simulink model "launch_gate_exp"  (R2022b)
settings: Solver=FixedStepDiscrete  StartTime=0.0  StopTime=5  FixedStep=0.001  RelTol=1e-3
InitFcn:
  | if ~exist('P','var') || ~isfield(P,'gate_version'), P=gate_params(launch_tcs_params()); end
model workspace (MAT data in the model file):
  w_2 : Simulink.Parameter (value not decoded)
undefined symbols (not defined in the file): A, a, B, b, C, D, DiscIntNeverNeededParam, Iz, K, k1, K1, k2, K2, L1, L2, m, magnitude, Phi, Sample_time, Steer_Ratio
libraries: simulink x26, slpidlib x13, Solver_SF x1, dsparch4 x1
(part 4 of 7)

== system launch_gate_exp/驱动防滑模块/Subsystem1 ==
  lamda2 : Inport
  p : Inport  Port=2
  i : Inport  Port=3
  b : Inport  Port=4
  Constant : Constant  Value=0.2
  PID Controller : slpidlib/PID Controller  Controller=PI  Form=Parallel  TimeDomain=Discrete-time  UseExternalTs=off  SampleTime=-1  IntegratorMethod=Forward Euler  FilterMethod=Forward Euler  ControllerParametersSource=external  P=5000  I=3000  UseKiTs=off  D=0  N=100  UseFilter=on  TunerSelectOption=Transfer Function Based (PID Tuner App)  InitialConditionSource=internal  InitialConditionForIntegrator=0  InitialConditionForFilter=0  DifferentiatorICPrevScaledInput=0  ExternalReset=none  TrackingMode=off  Kt=1  LimitOutput=on  SatLimitsSource=internal  UpperSaturationLimit=0  LowerSaturationLimit=-30000  LinearizeAsGain=on  AntiWindupMode=clamping  Kb=1  LimitIntegrator=off  UpperIntegratorSaturationLimit=inf  LowerIntegratorSaturationLimit=-inf  POutMin=[]  POutMax=[]  IOutMin=[]  IOutMax=[]  DOutMin=[]  DOutMax=[]  NOutMin=[]  NOutMax=[]  SumOutMin=[]  SumOutMax=[]  SaturationOutMin=[]  SaturationOutMax=[]  PParamMin=[]  PParamMax=[]  IParamMin=[]  IParamMax=[]  DParamMin=[]  DParamMax=[]  NParamMin=[]  NParamMax=[]  KbParamMin=[]  KbParamMax=[]  KtParamMin=[]  KtParamMax=[]  KbOutMin=[]  KbOutMax=[]  KtOutMin=[]  KtOutMax=[]  IntegratorOutMin=[]  IntegratorOutMax=[]  FilterOutMin=[]  FilterOutMax=[]  SumI1OutMin=[]  SumI1OutMax=[]  SumI2OutMin=[]  SumI2OutMax=[]  SumI3OutMin=[]  SumI3OutMax=[]  SumI4OutMin=[]  SumI4OutMax=[]  SumDOutMin=[]  SumDOutMax=[]  DifferentiatorOutMin=[]  DifferentiatorOutMax=[]  FilterDiffOutCoefMin=[]  FilterDiffOutCoefMax=[]  ReciprocalOutMin=[]  ReciprocalOutMax=[]  SumDenOutMin=[]  SumDenOutMax=[]  SumNumOutMin=[]  SumNumOutMax=[]  DivideOutMin=[]  DivideOutMax=[]  UdiffTsProdOutMin=[]  UdiffTsProdOutMax=[]  NTsProdOutMin=[]  NTsProdOutMax=[]  UintegralTsProdOutMin=[]  UintegralTsProdOutMax=[]  UngainTsProdOutMin=[]  UngainTsProdOutMax=[]  ClampingZeroOutDataTypeStr=Inherit: Inherit via back propagation  ClampingZeroOutMin=[]  ClampingZeroOutMax=[]  FilterDenConstantOutDataTypeStr=Inherit: Inherit via back propagation  FilterDenConstantOutMin=[]  FilterDenConstantOutMax=[]  PCopyOutDataTypeStr=Inherit: Inherit via back propagation  PCopyOutMin=[]  PCopyOutMax=[]  NCopyOutDataTypeStr=Inherit: Inherit via back propagation  NCopyOutMin=[]  NCopyOutMax=[]  IntegratorContinuousStateAttributes=''  IntegratorStateMustResolveToSignalObject=off  IntegratorRTWStateStorageClass=Auto  FilterContinuousStateAttributes=''  FilterStateMustResolveToSignalObject=off  FilterRTWStateStorageClass=Auto  ParallelPVariant=ExternalParameters  IdealPVariant=Disabled  IVariant=ExternalParameters  DVariant=Disabled  IntegratorVariant=Discrete  SatVariant=Enabled  AWVariant=DiscClampingParallel  PCopyVariant=Disabled  TRVariant=Disabled  FdbkBlocksVariant=Forward  IdealPFdbkVariant=Disabled  SatFdbkVariant=Disabled  DerivativeFilterVariant=Disabled  NVariant=Disabled  NCopyVariant=Disabled_SignalSpec  FilterICVariant=Disabled  IntegratorICVariant=InternalICs  ExternalResetVariant=Disabled  TRSumVariant=Passthrough  SumFdbkVariant=Disabled  SumVariant=Sum_PI  TsampFilterVariant=InternalTs  TsampNgainVariant=Passthrough  TsampIntegralVariant=Passthrough  ExternalSaturationOutDataTypeStr=Inherit: Same as second input
  Saturation : Saturate  UpperLimit=30000  LowerLimit=-99999
  Sum4 : Sum  Inputs=|+-
  dT1 : Outport
  wires:
  i/1 -> PID Controller/3
  p/1 -> PID Controller/2
  PID Controller/1 -> Saturation/1  "dT1"
  lamda2/1 -> Sum4/2
  Sum4/1 -> PID Controller/1
  Saturation/1 -> dT1/1
  Constant/1 -> Sum4/1

== system launch_gate_exp/驱动防滑模块/Subsystem2 ==
  lamda3 : Inport
  p : Inport  Port=2
  i : Inport  Port=3
  b : Inport  Port=4
  Constant : Constant  Value=0.2
  PID Controller : slpidlib/PID Controller  Controller=PI  Form=Parallel  TimeDomain=Discrete-time  UseExternalTs=off  SampleTime=-1  IntegratorMethod=Forward Euler  FilterMethod=Forward Euler  ControllerParametersSource=external  P=5000  I=3000  UseKiTs=off  D=0  N=100  UseFilter=on  TunerSelectOption=Transfer Function Based (PID Tuner App)  InitialConditionSource=internal  InitialConditionForIntegrator=0  InitialConditionForFilter=0  DifferentiatorICPrevScaledInput=0  ExternalReset=none  TrackingMode=off  Kt=1  LimitOutput=on  SatLimitsSource=internal  UpperSaturationLimit=0  LowerSaturationLimit=-50000  LinearizeAsGain=on  AntiWindupMode=clamping  Kb=1  LimitIntegrator=off  UpperIntegratorSaturationLimit=inf  LowerIntegratorSaturationLimit=-inf  POutMin=[]  POutMax=[]  IOutMin=[]  IOutMax=[]  DOutMin=[]  DOutMax=[]  NOutMin=[]  NOutMax=[]  SumOutMin=[]  SumOutMax=[]  SaturationOutMin=[]  SaturationOutMax=[]  PParamMin=[]  PParamMax=[]  IParamMin=[]  IParamMax=[]  DParamMin=[]  DParamMax=[]  NParamMin=[]  NParamMax=[]  KbParamMin=[]  KbParamMax=[]  KtParamMin=[]  KtParamMax=[]  KbOutMin=[]  KbOutMax=[]  KtOutMin=[]  KtOutMax=[]  IntegratorOutMin=[]  IntegratorOutMax=[]  FilterOutMin=[]  FilterOutMax=[]  SumI1OutMin=[]  SumI1OutMax=[]  SumI2OutMin=[]  SumI2OutMax=[]  SumI3OutMin=[]  SumI3OutMax=[]  SumI4OutMin=[]  SumI4OutMax=[]  SumDOutMin=[]  SumDOutMax=[]  DifferentiatorOutMin=[]  DifferentiatorOutMax=[]  FilterDiffOutCoefMin=[]  FilterDiffOutCoefMax=[]  ReciprocalOutMin=[]  ReciprocalOutMax=[]  SumDenOutMin=[]  SumDenOutMax=[]  SumNumOutMin=[]  SumNumOutMax=[]  DivideOutMin=[]  DivideOutMax=[]  UdiffTsProdOutMin=[]  UdiffTsProdOutMax=[]  NTsProdOutMin=[]  NTsProdOutMax=[]  UintegralTsProdOutMin=[]  UintegralTsProdOutMax=[]  UngainTsProdOutMin=[]  UngainTsProdOutMax=[]  ClampingZeroOutDataTypeStr=Inherit: Inherit via back propagation  ClampingZeroOutMin=[]  ClampingZeroOutMax=[]  FilterDenConstantOutDataTypeStr=Inherit: Inherit via back propagation  FilterDenConstantOutMin=[]  FilterDenConstantOutMax=[]  PCopyOutDataTypeStr=Inherit: Inherit via back propagation  PCopyOutMin=[]  PCopyOutMax=[]  NCopyOutDataTypeStr=Inherit: Inherit via back propagation  NCopyOutMin=[]  NCopyOutMax=[]  IntegratorContinuousStateAttributes=''  IntegratorStateMustResolveToSignalObject=off  IntegratorRTWStateStorageClass=Auto  FilterContinuousStateAttributes=''  FilterStateMustResolveToSignalObject=off  FilterRTWStateStorageClass=Auto  ParallelPVariant=ExternalParameters  IdealPVariant=Disabled  IVariant=ExternalParameters  DVariant=Disabled  IntegratorVariant=Discrete  SatVariant=Enabled  AWVariant=DiscClampingParallel  PCopyVariant=Disabled  TRVariant=Disabled  FdbkBlocksVariant=Forward  IdealPFdbkVariant=Disabled  SatFdbkVariant=Disabled  DerivativeFilterVariant=Disabled  NVariant=Disabled  NCopyVariant=Disabled_SignalSpec  FilterICVariant=Disabled  IntegratorICVariant=InternalICs  ExternalResetVariant=Disabled  TRSumVariant=Passthrough  SumFdbkVariant=Disabled  SumVariant=Sum_PI  TsampFilterVariant=InternalTs  TsampNgainVariant=Passthrough  TsampIntegralVariant=Passthrough  ExternalSaturationOutDataTypeStr=Inherit: Same as second input
  Saturation : Saturate  UpperLimit=30000  LowerLimit=-99999
  Sum4 : Sum  Inputs=|+-
  dT1 : Outport
  wires:
  Sum4/1 -> PID Controller/1
  lamda3/1 -> Sum4/2
  PID Controller/1 -> Saturation/1  "dT1"
  p/1 -> PID Controller/2
  i/1 -> PID Controller/3
  Saturation/1 -> dT1/1
  Constant/1 -> Sum4/1

== system launch_gate_exp/驱动防滑模块/Subsystem3 ==
  lamda4 : Inport
  p : Inport  Port=2
  i : Inport  Port=3
  b : Inport  Port=4
  Constant : Constant  Value=0.2
  PID Controller : slpidlib/PID Controller  Controller=PI  Form=Parallel  TimeDomain=Discrete-time  UseExternalTs=off  SampleTime=-1  IntegratorMethod=Forward Euler  FilterMethod=Forward Euler  ControllerParametersSource=external  P=5000  I=3000  UseKiTs=off  D=0  N=100  UseFilter=on  TunerSelectOption=Transfer Function Based (PID Tuner App)  InitialConditionSource=internal  InitialConditionForIntegrator=0  InitialConditionForFilter=0  DifferentiatorICPrevScaledInput=0  ExternalReset=none  TrackingMode=off  Kt=1  LimitOutput=on  SatLimitsSource=internal  UpperSaturationLimit=0  LowerSaturationLimit=-50000  LinearizeAsGain=on  AntiWindupMode=clamping  Kb=1  LimitIntegrator=off  UpperIntegratorSaturationLimit=inf  LowerIntegratorSaturationLimit=-inf  POutMin=[]  POutMax=[]  IOutMin=[]  IOutMax=[]  DOutMin=[]  DOutMax=[]  NOutMin=[]  NOutMax=[]  SumOutMin=[]  SumOutMax=[]  SaturationOutMin=[]  SaturationOutMax=[]  PParamMin=[]  PParamMax=[]  IParamMin=[]  IParamMax=[]  DParamMin=[]  DParamMax=[]  NParamMin=[]  NParamMax=[]  KbParamMin=[]  KbParamMax=[]  KtParamMin=[]  KtParamMax=[]  KbOutMin=[]  KbOutMax=[]  KtOutMin=[]  KtOutMax=[]  IntegratorOutMin=[]  IntegratorOutMax=[]  FilterOutMin=[]  FilterOutMax=[]  SumI1OutMin=[]  SumI1OutMax=[]  SumI2OutMin=[]  SumI2OutMax=[]  SumI3OutMin=[]  SumI3OutMax=[]  SumI4OutMin=[]  SumI4OutMax=[]  SumDOutMin=[]  SumDOutMax=[]  DifferentiatorOutMin=[]  DifferentiatorOutMax=[]  FilterDiffOutCoefMin=[]  FilterDiffOutCoefMax=[]  ReciprocalOutMin=[]  ReciprocalOutMax=[]  SumDenOutMin=[]  SumDenOutMax=[]  SumNumOutMin=[]  SumNumOutMax=[]  DivideOutMin=[]  DivideOutMax=[]  UdiffTsProdOutMin=[]  UdiffTsProdOutMax=[]  NTsProdOutMin=[]  NTsProdOutMax=[]  UintegralTsProdOutMin=[]  UintegralTsProdOutMax=[]  UngainTsProdOutMin=[]  UngainTsProdOutMax=[]  ClampingZeroOutDataTypeStr=Inherit: Inherit via back propagation  ClampingZeroOutMin=[]  ClampingZeroOutMax=[]  FilterDenConstantOutDataTypeStr=Inherit: Inherit via back propagation  FilterDenConstantOutMin=[]  FilterDenConstantOutMax=[]  PCopyOutDataTypeStr=Inherit: Inherit via back propagation  PCopyOutMin=[]  PCopyOutMax=[]  NCopyOutDataTypeStr=Inherit: Inherit via back propagation  NCopyOutMin=[]  NCopyOutMax=[]  IntegratorContinuousStateAttributes=''  IntegratorStateMustResolveToSignalObject=off  IntegratorRTWStateStorageClass=Auto  FilterContinuousStateAttributes=''  FilterStateMustResolveToSignalObject=off  FilterRTWStateStorageClass=Auto  ParallelPVariant=ExternalParameters  IdealPVariant=Disabled  IVariant=ExternalParameters  DVariant=Disabled  IntegratorVariant=Discrete  SatVariant=Enabled  AWVariant=DiscClampingParallel  PCopyVariant=Disabled  TRVariant=Disabled  FdbkBlocksVariant=Forward  IdealPFdbkVariant=Disabled  SatFdbkVariant=Disabled  DerivativeFilterVariant=Disabled  NVariant=Disabled  NCopyVariant=Disabled_SignalSpec  FilterICVariant=Disabled  IntegratorICVariant=InternalICs  ExternalResetVariant=Disabled  TRSumVariant=Passthrough  SumFdbkVariant=Disabled  SumVariant=Sum_PI  TsampFilterVariant=InternalTs  TsampNgainVariant=Passthrough  TsampIntegralVariant=Passthrough  ExternalSaturationOutDataTypeStr=Inherit: Same as second input
  Saturation : Saturate  UpperLimit=30000  LowerLimit=-99999
  Sum4 : Sum  Inputs=|+-
  dT1 : Outport
  wires:
  i/1 -> PID Controller/3
  p/1 -> PID Controller/2
  PID Controller/1 -> Saturation/1  "dT1"
  lamda4/1 -> Sum4/2
  Sum4/1 -> PID Controller/1
  Saturation/1 -> dT1/1
  Constant/1 -> Sum4/1

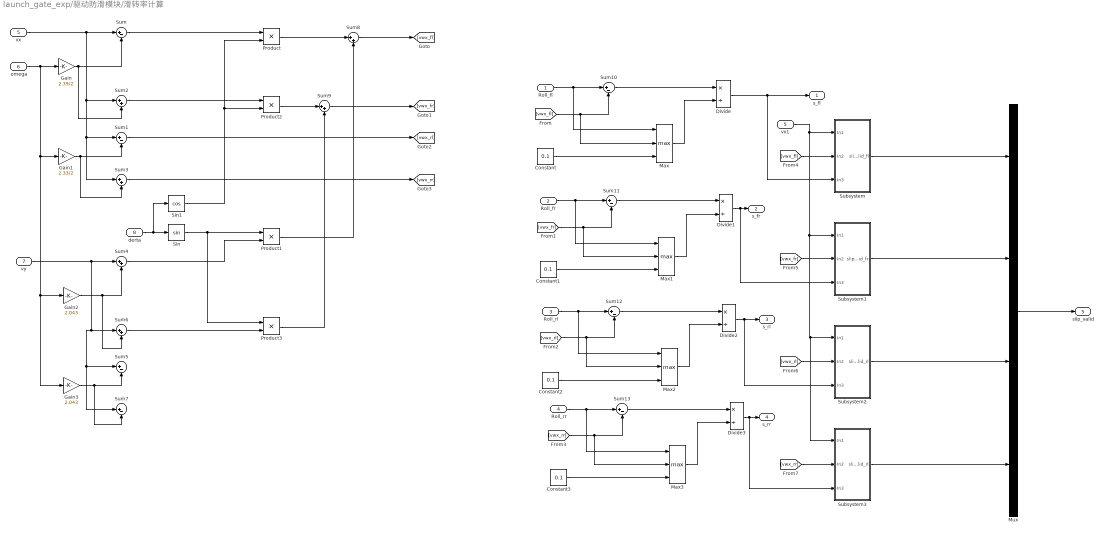
== system launch_gate_exp/驱动防滑模块/滑转率计算 ==
  Roll_fl : Inport
  Roll_fr : Inport  Port=2
  Roll_rl : Inport  Port=3
  Roll_rr : Inport  Port=4
  vx : Inport  Port=5
  omega : Inport  Port=6
  vy : Inport  Port=7
  derta : Inport  Port=8
  Constant{,1..3} (4 alike) : Constant  Value=0.1
  Divide{,1..3} (4 alike) : Product  Inputs=*/
  Gain : Gain  Gain=2.39/2
  Gain1 : Gain  Gain=2.33/2
  Gain2 : Gain  Gain=2.043
  Gain3 : Gain  Gain=2.043
  Max{,1..3} (4 alike) : MinMax  Function=max  Inputs=3
  Mux : Mux
  Product{,1..3} (4 alike) : Product
  Sin : Trigonometry
  Sin1 : Trigonometry  Operator=cos
  Subsystem : Subsystem
  Subsystem1 : Subsystem
  Subsystem2 : Subsystem
  Subsystem3 : Subsystem
  Sum{,1,5,7,10..13} (8 alike) : Sum  Inputs=|+-
  Sum{2..4,6,8..9} (6 alike) : Sum  Inputs=|++
  vx1 : InportShadow  Port=5
  s_fl : Outport
  s_fr : Outport  Port=2
  s_rl : Outport  Port=3
  s_rr : Outport  Port=4
  slip_valid : Outport  Port=5
  wires:
  vx/1 -> Sum3/1, Sum1/1, Sum2/1, Sum/1
  Gain/1 -> Sum2/2, Sum/2
  Gain1/1 -> Sum3/2, Sum1/2
  Gain3/1 -> Sum5/2, Sum7/2
  Gain2/1 -> Sum4/2, Sum6/2
  omega/1 -> Gain3/1, Gain2/1, Gain1/1, Gain/1
  vy/1 -> Sum4/1, Sum5/1, Sum7/1, Sum6/1
  derta/1 -> Sin1/1, Sin/1
  Sum/1 -> Product/1
  Sin1/1 -> Product2/2, Product/2
  Product/1 -> Sum8/1
  Sin/1 -> Product3/1, Product1/1
  Sum4/1 -> Product1/2
  Product1/1 -> Sum8/2
  Sum8/1 -> [vwx_fl]
  Sum2/1 -> Product2/1
  Product2/1 -> Sum9/1
  Sum6/1 -> Product3/2
  Product3/1 -> Sum9/2
  Sum9/1 -> [vwx_fr]
  Sum1/1 -> [vwx_rl]
  Sum3/1 -> [vwx_rr]
  Roll_fl/1 -> Max/1, Sum10/1
  [vwx_fl] -> Max/2, Sum10/2
  Sum10/1 -> Divide/1
  Constant/1 -> Max/3
  Max/1 -> Divide/2
  Divide/1 -> Subsystem/3(In3), s_fl/1
  Divide1/1 -> Subsystem1/3(In3), s_fr/1
  Max1/1 -> Divide1/2
  Constant1/1 -> Max1/3
  Sum11/1 -> Divide1/1
  [vwx_fr] -> Sum11/2, Max1/2
  Roll_fr/1 -> Sum11/1, Max1/1
  Roll_rl/1 -> Max2/1, Sum12/1
  [vwx_rl] -> Max2/2, Sum12/2
  Sum12/1 -> Divide2/1
  Constant2/1 -> Max2/3
  Max2/1 -> Divide2/2
  Divide2/1 -> Subsystem2/3(In3), s_rl/1
  Divide3/1 -> Subsystem3/3(In3), s_rr/1
  Max3/1 -> Divide3/2
  Constant3/1 -> Max3/3
  Sum13/1 -> Divide3/1
  [vwx_rr] -> Sum13/2, Max3/2
  Roll_rr/1 -> Sum13/1, Max3/1
  vx1/1 -> Subsystem3/1(In1), Subsystem2/1(In1), Subsystem1/1(In1), Subsystem/1(In1)
  [vwx_fl] -> Subsystem/2(In2)
  [vwx_fr] -> Subsystem1/2(In2)
  [vwx_rl] -> Subsystem2/2(In2)
  [vwx_rr] -> Subsystem3/2(In2)
  Subsystem/1(slip_valid_fl) -> Mux/1
  Subsystem1/1(slip_valid_fr) -> Mux/2
  Subsystem2/1(slip_valid_rl) -> Mux/3
  Subsystem3/1(slip_valid_rl) -> Mux/4
  Mux/1 -> slip_valid/1

== system launch_gate_exp/Dugoff轮胎模型/alpha_lamda/alpha ==
  vx : Inport
  vy : Inport  Port=2
  wz : Inport  Port=3
  delta_fl : Inport  Port=4
  delta_fr : Inport  Port=5
  Gain{,1..3} (4 alike) : Gain  Gain=-1
  fl : Subsystem
  fr : Subsystem
  rl : Subsystem
  rr : Subsystem
  alpha_fl : Outport
  alpha_fr : Outport  Port=2
  alpha_rl : Outport  Port=3
  alpha_rr : Outport  Port=4
  wires:
  delta_fr/1 -> fr/4(delta_fr)
  delta_fl/1 -> fl/4(delta_fl)
  vy/1 -> rl/2(vy), fl/2(vy), fr/2(vy), rr/2(vy)
  vx/1 -> rl/1(vx), fl/1(vx), fr/1(vx), rr/1(vx)
  wz/1 -> rl/3(wz), fr/3(wz), rr/3(wz), fl/3(wz)
  fl/1(alpha_fl) -> Gain/1
  Gain/1 -> alpha_fl/1
  rl/1(alpha_rl) -> Gain1/1
  Gain1/1 -> alpha_rl/1
  fr/1(alpha_fr) -> Gain2/1
  Gain2/1 -> alpha_fr/1
  rr/1(alpha_rr) -> Gain3/1
  Gain3/1 -> alpha_rr/1

== system launch_gate_exp/Dugoff轮胎模型/alpha_lamda/lamda ==
  vx : Inport
  vy : Inport  Port=2
  wz : Inport  Port=3
  delta_fl : Inport  Port=4
  delta_fr : Inport  Port=5
  w_fl : Inport  Port=6
  w_fr : Inport  Port=7
  w_rl : Inport  Port=8
  w_rr : Inport  Port=9
  fl : Subsystem
  fr : Subsystem
  rl : Subsystem
  rr : Subsystem
  lamda_fl : Outport
  lamda_fr : Outport  Port=2
  lamda_rl : Outport  Port=3
  lamda_rr : Outport  Port=4
  wires:
  fr/1(lamda_fr) -> lamda_fr/1
  rr/1(lamda_rr) -> lamda_rr/1
  w_rl/1 -> rl/1(w_rl)
  w_rr/1 -> rr/1(w_rr)
  w_fr/1 -> fr/1(w_fr)
  delta_fr/1 -> fr/5(delta_fr)
  delta_fl/1 -> fl/5(delta_fl)
  vy/1 -> fl/4(vy), fr/4(vy)
  vx/1 -> fl/3(vx), fr/3(vx), rr/3(vx), rl/3(vx)
  wz/1 -> fl/2(wz), fr/2(wz), rr/2(wz), rl/2(wz)
  w_fl/1 -> fl/1(w_fl)
  rl/1(lamda_rl) -> lamda_rl/1
  fl/1(lamda_fl) -> lamda_fl/1

== system launch_gate_exp/四轮转矩分配/下层轮胎力执行控制器/右前轮 ==
  FzR1 : Inport
  FxR1 : Inport  Port=2
  FyR1 : Inport  Port=3
  kappa_R1 : Inport  Port=4
  derta : Inport  Port=5
  Gain : Gain  Gain=0.834
  If : If  IfExpression=u1 > 52000  ElseIfExpressions=u1<18000
  If Action Subsystem : Subsystem  TreatAsAtomicUnit=on
  If Action Subsystem1 : Subsystem  TreatAsAtomicUnit=on
  If Action Subsystem2 : Subsystem  TreatAsAtomicUnit=on
  Merge : Merge  Inputs=3
  PID Controller : slpidlib/PID Controller  Controller=PID  Form=Parallel  TimeDomain=Discrete-time  UseExternalTs=off  SampleTime=-1  IntegratorMethod=Forward Euler  FilterMethod=Forward Euler  ControllerParametersSource=internal  P=3500  I=3000  UseKiTs=off  D=0  N=100  UseFilter=on  TunerSelectOption=Transfer Function Based (PID Tuner App)  InitialConditionSource=internal  InitialConditionForIntegrator=0  InitialConditionForFilter=0  DifferentiatorICPrevScaledInput=0  ExternalReset=none  TrackingMode=off  Kt=1  LimitOutput=off  SatLimitsSource=internal  UpperSaturationLimit=inf  LowerSaturationLimit=-inf  LinearizeAsGain=on  AntiWindupMode=none  Kb=1  LimitIntegrator=off  UpperIntegratorSaturationLimit=inf  LowerIntegratorSaturationLimit=-inf  POutMin=[]  POutMax=[]  IOutMin=[]  IOutMax=[]  DOutMin=[]  DOutMax=[]  NOutMin=[]  NOutMax=[]  SumOutMin=[]  SumOutMax=[]  SaturationOutMin=[]  SaturationOutMax=[]  PParamMin=[]  PParamMax=[]  IParamMin=[]  IParamMax=[]  DParamMin=[]  DParamMax=[]  NParamMin=[]  NParamMax=[]  KbParamMin=[]  KbParamMax=[]  KtParamMin=[]  KtParamMax=[]  KbOutMin=[]  KbOutMax=[]  KtOutMin=[]  KtOutMax=[]  IntegratorOutMin=[]  IntegratorOutMax=[]  FilterOutMin=[]  FilterOutMax=[]  SumI1OutMin=[]  SumI1OutMax=[]  SumI2OutMin=[]  SumI2OutMax=[]  SumI3OutMin=[]  SumI3OutMax=[]  SumI4OutMin=[]  SumI4OutMax=[]  SumDOutMin=[]  SumDOutMax=[]  DifferentiatorOutMin=[]  DifferentiatorOutMax=[]  FilterDiffOutCoefMin=[]  FilterDiffOutCoefMax=[]  ReciprocalOutMin=[]  ReciprocalOutMax=[]  SumDenOutMin=[]  SumDenOutMax=[]  SumNumOutMin=[]  SumNumOutMax=[]  DivideOutMin=[]  DivideOutMax=[]  UdiffTsProdOutMin=[]  UdiffTsProdOutMax=[]  NTsProdOutMin=[]  NTsProdOutMax=[]  UintegralTsProdOutMin=[]  UintegralTsProdOutMax=[]  UngainTsProdOutMin=[]  UngainTsProdOutMax=[]  ClampingZeroOutDataTypeStr=Inherit: Inherit via back propagation  ClampingZeroOutMin=[]  ClampingZeroOutMax=[]  FilterDenConstantOutDataTypeStr=Inherit: Inherit via back propagation  FilterDenConstantOutMin=[]  FilterDenConstantOutMax=[]  PCopyOutDataTypeStr=Inherit: Inherit via back propagation  PCopyOutMin=[]  PCopyOutMax=[]  NCopyOutDataTypeStr=Inherit: Inherit via back propagation  NCopyOutMin=[]  NCopyOutMax=[]  IntegratorContinuousStateAttributes=''  IntegratorStateMustResolveToSignalObject=off  IntegratorRTWStateStorageClass=Auto  FilterContinuousStateAttributes=''  FilterStateMustResolveToSignalObject=off  FilterRTWStateStorageClass=Auto  ParallelPVariant=InternalParameters  IdealPVariant=Disabled  IVariant=InternalParameters  DVariant=InternalParameters  IntegratorVariant=Discrete  SatVariant=Disabled  AWVariant=Passthrough  PCopyVariant=Disabled  TRVariant=Disabled  FdbkBlocksVariant=Forward  IdealPFdbkVariant=Disabled  SatFdbkVariant=Disabled  DerivativeFilterVariant=ForwardEulerFilter  NVariant=InternalParameters  NCopyVariant=Disabled  FilterICVariant=InternalICsFilter  IntegratorICVariant=InternalICs  ExternalResetVariant=Disabled  TRSumVariant=Passthrough  SumFdbkVariant=Disabled  SumVariant=Sum_PID  TsampFilterVariant=InternalTs  TsampNgainVariant=Passthrough  TsampIntegralVariant=Passthrough  ExternalSaturationOutDataTypeStr=Inherit: Same as second input
  Product : Product
  Product1 : Product
  Saturation1 : Saturate  UpperLimit=1100*63.52  LowerLimit=0
  Sin : Trigonometry
  Sin1 : Trigonometry  Operator=cos
  Sum : Sum  Inputs=|++
  Sum1 : Sum  Inputs=|+-
  Sum2 : Sum  Inputs=|++
  Torque2 : Scope  NumInputPorts=2
  kappa2 : Scope  NumInputPorts=2
  Out1 : Outport
  wires:
  If Action Subsystem1/1(kappa_d) -> Merge/1
  If Action Subsystem2/1(kappa_d) -> Merge/3
  Product1/1 -> Sum/1
  Gain/1 -> Sum2/2
  Product/1 -> Sum/2
  Sin1/1 -> Product1/2
  If/3 -> If Action Subsystem2/Action
  derta/1 -> Sin/1, Sin1/1
  Sum/1 -> Gain/1
  kappa_R1/1 -> kappa2/2, Sum1/2
  FzR1/1 -> If/1
  If Action Subsystem/1(kappa_d) -> Merge/2
  If/2 -> If Action Subsystem/Action
  FyR1/1 -> Product/1
  Sum2/1 -> Torque2/2, Saturation1/1
  Sin/1 -> Product/2
  FxR1/1 -> If Action Subsystem/1(Fx), If Action Subsystem1/1(Fx), If Action Subsystem2/1(Fx), Product1/1
  If/1 -> If Action Subsystem1/Action
  Saturation1/1 -> Out1/1
  Sum1/1 -> PID Controller/1
  Merge/1 -> kappa2/1, Sum1/1
  PID Controller/1 -> Torque2/1, Sum2/1

== system launch_gate_exp/四轮转矩分配/下层轮胎力执行控制器/右后轮 ==
  FzR2 : Inport
  FxR2 : Inport  Port=2
  kappa_R2 : Inport  Port=3
  Gain : Gain  Gain=0.94
  If : If  IfExpression=u1 > 69000  ElseIfExpressions=u1<35000
  If Action Subsystem : Subsystem  TreatAsAtomicUnit=on
  If Action Subsystem1 : Subsystem  TreatAsAtomicUnit=on
  If Action Subsystem2 : Subsystem  TreatAsAtomicUnit=on
  Merge : Merge  Inputs=3
  PID Controller : slpidlib/PID Controller  Controller=PID  Form=Parallel  TimeDomain=Discrete-time  UseExternalTs=off  SampleTime=-1  IntegratorMethod=Forward Euler  FilterMethod=Forward Euler  ControllerParametersSource=internal  P=3500  I=3000  UseKiTs=off  D=0  N=100  UseFilter=on  TunerSelectOption=Transfer Function Based (PID Tuner App)  InitialConditionSource=internal  InitialConditionForIntegrator=0  InitialConditionForFilter=0  DifferentiatorICPrevScaledInput=0  ExternalReset=none  TrackingMode=off  Kt=1  LimitOutput=off  SatLimitsSource=internal  UpperSaturationLimit=inf  LowerSaturationLimit=-inf  LinearizeAsGain=on  AntiWindupMode=none  Kb=1  LimitIntegrator=off  UpperIntegratorSaturationLimit=inf  LowerIntegratorSaturationLimit=-inf  POutMin=[]  POutMax=[]  IOutMin=[]  IOutMax=[]  DOutMin=[]  DOutMax=[]  NOutMin=[]  NOutMax=[]  SumOutMin=[]  SumOutMax=[]  SaturationOutMin=[]  SaturationOutMax=[]  PParamMin=[]  PParamMax=[]  IParamMin=[]  IParamMax=[]  DParamMin=[]  DParamMax=[]  NParamMin=[]  NParamMax=[]  KbParamMin=[]  KbParamMax=[]  KtParamMin=[]  KtParamMax=[]  KbOutMin=[]  KbOutMax=[]  KtOutMin=[]  KtOutMax=[]  IntegratorOutMin=[]  IntegratorOutMax=[]  FilterOutMin=[]  FilterOutMax=[]  SumI1OutMin=[]  SumI1OutMax=[]  SumI2OutMin=[]  SumI2OutMax=[]  SumI3OutMin=[]  SumI3OutMax=[]  SumI4OutMin=[]  SumI4OutMax=[]  SumDOutMin=[]  SumDOutMax=[]  DifferentiatorOutMin=[]  DifferentiatorOutMax=[]  FilterDiffOutCoefMin=[]  FilterDiffOutCoefMax=[]  ReciprocalOutMin=[]  ReciprocalOutMax=[]  SumDenOutMin=[]  SumDenOutMax=[]  SumNumOutMin=[]  SumNumOutMax=[]  DivideOutMin=[]  DivideOutMax=[]  UdiffTsProdOutMin=[]  UdiffTsProdOutMax=[]  NTsProdOutMin=[]  NTsProdOutMax=[]  UintegralTsProdOutMin=[]  UintegralTsProdOutMax=[]  UngainTsProdOutMin=[]  UngainTsProdOutMax=[]  ClampingZeroOutDataTypeStr=Inherit: Inherit via back propagation  ClampingZeroOutMin=[]  ClampingZeroOutMax=[]  FilterDenConstantOutDataTypeStr=Inherit: Inherit via back propagation  FilterDenConstantOutMin=[]  FilterDenConstantOutMax=[]  PCopyOutDataTypeStr=Inherit: Inherit via back propagation  PCopyOutMin=[]  PCopyOutMax=[]  NCopyOutDataTypeStr=Inherit: Inherit via back propagation  NCopyOutMin=[]  NCopyOutMax=[]  IntegratorContinuousStateAttributes=''  IntegratorStateMustResolveToSignalObject=off  IntegratorRTWStateStorageClass=Auto  FilterContinuousStateAttributes=''  FilterStateMustResolveToSignalObject=off  FilterRTWStateStorageClass=Auto  ParallelPVariant=InternalParameters  IdealPVariant=Disabled  IVariant=InternalParameters  DVariant=InternalParameters  IntegratorVariant=Discrete  SatVariant=Disabled  AWVariant=Passthrough  PCopyVariant=Disabled  TRVariant=Disabled  FdbkBlocksVariant=Forward  IdealPFdbkVariant=Disabled  SatFdbkVariant=Disabled  DerivativeFilterVariant=ForwardEulerFilter  NVariant=InternalParameters  NCopyVariant=Disabled  FilterICVariant=InternalICsFilter  IntegratorICVariant=InternalICs  ExternalResetVariant=Disabled  TRSumVariant=Passthrough  SumFdbkVariant=Disabled  SumVariant=Sum_PID  TsampFilterVariant=InternalTs  TsampNgainVariant=Passthrough  TsampIntegralVariant=Passthrough  ExternalSaturationOutDataTypeStr=Inherit: Same as second input
  Saturation3 : Saturate  UpperLimit=1800*80.4  LowerLimit=0
  Sum1 : Sum  Inputs=|+-
  Sum2 : Sum  Inputs=|++
  Torque4 : Scope  NumInputPorts=2
  kappa4 : Scope  NumInputPorts=2
  Out1 : Outport
  wires:
  If/1 -> If Action Subsystem1/Action
  If/2 -> If Action Subsystem/Action
  If Action Subsystem/1(kappa_d) -> Merge/2
  FzR2/1 -> If/1
  Sum1/1 -> PID Controller/1
  FxR2/1 -> If Action Subsystem2/1(Fx), Gain/1, If Action Subsystem1/1(Fx), If Action Subsystem/1(Fx)
  If/3 -> If Action Subsystem2/Action
  Gain/1 -> Sum2/2
  If Action Subsystem2/1(kappa_d) -> Merge/3
  If Action Subsystem1/1(kappa_d) -> Merge/1
  Saturation3/1 -> Out1/1
  Sum2/1 -> Torque4/2, Saturation3/1
  kappa_R2/1 -> kappa4/2, Sum1/2
  Merge/1 -> kappa4/1, Sum1/1
  PID Controller/1 -> Torque4/1, Sum2/1

== system launch_gate_exp/四轮转矩分配/下层轮胎力执行控制器/左前轮 ==
  FzL1 : Inport
  FxL1 : Inport  Port=2
  FyL1 : Inport  Port=3
  kappa_L1 : Inport  Port=4
  derta : Inport  Port=5
  Gain : Gain  Gain=0.834
  If : If  IfExpression=u1 > 52000  ElseIfExpressions=u1<18000
  If Action Subsystem : Subsystem  TreatAsAtomicUnit=on
  If Action Subsystem1 : Subsystem  TreatAsAtomicUnit=on
  If Action Subsystem2 : Subsystem  TreatAsAtomicUnit=on
  Merge : Merge  Inputs=3
  PID Controller : slpidlib/PID Controller  Controller=PID  Form=Parallel  TimeDomain=Discrete-time  UseExternalTs=off  SampleTime=-1  IntegratorMethod=Forward Euler  FilterMethod=Forward Euler  ControllerParametersSource=internal  P=3500  I=3000  UseKiTs=off  D=0  N=100  UseFilter=on  TunerSelectOption=Transfer Function Based (PID Tuner App)  InitialConditionSource=internal  InitialConditionForIntegrator=0  InitialConditionForFilter=0  DifferentiatorICPrevScaledInput=0  ExternalReset=none  TrackingMode=off  Kt=1  LimitOutput=off  SatLimitsSource=internal  UpperSaturationLimit=inf  LowerSaturationLimit=-inf  LinearizeAsGain=on  AntiWindupMode=none  Kb=1  LimitIntegrator=off  UpperIntegratorSaturationLimit=inf  LowerIntegratorSaturationLimit=-inf  POutMin=[]  POutMax=[]  IOutMin=[]  IOutMax=[]  DOutMin=[]  DOutMax=[]  NOutMin=[]  NOutMax=[]  SumOutMin=[]  SumOutMax=[]  SaturationOutMin=[]  SaturationOutMax=[]  PParamMin=[]  PParamMax=[]  IParamMin=[]  IParamMax=[]  DParamMin=[]  DParamMax=[]  NParamMin=[]  NParamMax=[]  KbParamMin=[]  KbParamMax=[]  KtParamMin=[]  KtParamMax=[]  KbOutMin=[]  KbOutMax=[]  KtOutMin=[]  KtOutMax=[]  IntegratorOutMin=[]  IntegratorOutMax=[]  FilterOutMin=[]  FilterOutMax=[]  SumI1OutMin=[]  SumI1OutMax=[]  SumI2OutMin=[]  SumI2OutMax=[]  SumI3OutMin=[]  SumI3OutMax=[]  SumI4OutMin=[]  SumI4OutMax=[]  SumDOutMin=[]  SumDOutMax=[]  DifferentiatorOutMin=[]  DifferentiatorOutMax=[]  FilterDiffOutCoefMin=[]  FilterDiffOutCoefMax=[]  ReciprocalOutMin=[]  ReciprocalOutMax=[]  SumDenOutMin=[]  SumDenOutMax=[]  SumNumOutMin=[]  SumNumOutMax=[]  DivideOutMin=[]  DivideOutMax=[]  UdiffTsProdOutMin=[]  UdiffTsProdOutMax=[]  NTsProdOutMin=[]  NTsProdOutMax=[]  UintegralTsProdOutMin=[]  UintegralTsProdOutMax=[]  UngainTsProdOutMin=[]  UngainTsProdOutMax=[]  ClampingZeroOutDataTypeStr=Inherit: Inherit via back propagation  ClampingZeroOutMin=[]  ClampingZeroOutMax=[]  FilterDenConstantOutDataTypeStr=Inherit: Inherit via back propagation  FilterDenConstantOutMin=[]  FilterDenConstantOutMax=[]  PCopyOutDataTypeStr=Inherit: Inherit via back propagation  PCopyOutMin=[]  PCopyOutMax=[]  NCopyOutDataTypeStr=Inherit: Inherit via back propagation  NCopyOutMin=[]  NCopyOutMax=[]  IntegratorContinuousStateAttributes=''  IntegratorStateMustResolveToSignalObject=off  IntegratorRTWStateStorageClass=Auto  FilterContinuousStateAttributes=''  FilterStateMustResolveToSignalObject=off  FilterRTWStateStorageClass=Auto  ParallelPVariant=InternalParameters  IdealPVariant=Disabled  IVariant=InternalParameters  DVariant=InternalParameters  IntegratorVariant=Discrete  SatVariant=Disabled  AWVariant=Passthrough  PCopyVariant=Disabled  TRVariant=Disabled  FdbkBlocksVariant=Forward  IdealPFdbkVariant=Disabled  SatFdbkVariant=Disabled  DerivativeFilterVariant=ForwardEulerFilter  NVariant=InternalParameters  NCopyVariant=Disabled  FilterICVariant=InternalICsFilter  IntegratorICVariant=InternalICs  ExternalResetVariant=Disabled  TRSumVariant=Passthrough  SumFdbkVariant=Disabled  SumVariant=Sum_PID  TsampFilterVariant=InternalTs  TsampNgainVariant=Passthrough  TsampIntegralVariant=Passthrough  ExternalSaturationOutDataTypeStr=Inherit: Same as second input
  Product : Product
  Product1 : Product
  Saturation1 : Saturate  UpperLimit=1100*63.52  LowerLimit=0
  Sin : Trigonometry
  Sin1 : Trigonometry  Operator=cos
  Sum : Sum  Inputs=|++
  Sum1 : Sum  Inputs=|+-
  Sum2 : Sum  Inputs=|++
  Torque : Scope  NumInputPorts=2
  kappa : Scope  NumInputPorts=2
  Out1 : Outport
  wires:
  If/1 -> If Action Subsystem1/Action
  FxL1/1 -> Product1/1, If Action Subsystem2/1(Fx), If Action Subsystem1/1(Fx), If Action Subsystem/1(Fx)
  Sin/1 -> Product/2
  Sum2/1 -> Torque/2, Saturation1/1
  FyL1/1 -> Product/1
  If/2 -> If Action Subsystem/Action
  If Action Subsystem/1(kappa_d) -> Merge/2
  FzL1/1 -> If/1
  kappa_L1/1 -> kappa/2, Sum1/2
  Sum1/1 -> PID Controller/1
  Sum/1 -> Gain/1
  derta/1 -> Sin1/1, Sin/1
  If/3 -> If Action Subsystem2/Action
  Sin1/1 -> Product1/2
  Merge/1 -> kappa/1, Sum1/1
  Product/1 -> Sum/2
  Gain/1 -> Sum2/2
  PID Controller/1 -> Torque/1, Sum2/1
  Product1/1 -> Sum/1
  If Action Subsystem2/1(kappa_d) -> Merge/3
  If Action Subsystem1/1(kappa_d) -> Merge/1
  Saturation1/1 -> Out1/1

== system launch_gate_exp/四轮转矩分配/下层轮胎力执行控制器/左后轮 ==
  FzL2 : Inport
  FxL2 : Inport  Port=2
  kappa_L2 : Inport  Port=3
  Gain : Gain  Gain=0.94
  If : If  IfExpression=u1 > 69000  ElseIfExpressions=u1<35000
  If Action Subsystem : Subsystem  TreatAsAtomicUnit=on
  If Action Subsystem1 : Subsystem  TreatAsAtomicUnit=on
  If Action Subsystem2 : Subsystem  TreatAsAtomicUnit=on
  Merge : Merge  Inputs=3
  PID Controller : slpidlib/PID Controller  Controller=PID  Form=Parallel  TimeDomain=Discrete-time  UseExternalTs=off  SampleTime=-1  IntegratorMethod=Forward Euler  FilterMethod=Forward Euler  ControllerParametersSource=internal  P=3500  I=3000  UseKiTs=off  D=0  N=100  UseFilter=on  TunerSelectOption=Transfer Function Based (PID Tuner App)  InitialConditionSource=internal  InitialConditionForIntegrator=0  InitialConditionForFilter=0  DifferentiatorICPrevScaledInput=0  ExternalReset=none  TrackingMode=off  Kt=1  LimitOutput=off  SatLimitsSource=internal  UpperSaturationLimit=inf  LowerSaturationLimit=-inf  LinearizeAsGain=on  AntiWindupMode=none  Kb=1  LimitIntegrator=off  UpperIntegratorSaturationLimit=inf  LowerIntegratorSaturationLimit=-inf  POutMin=[]  POutMax=[]  IOutMin=[]  IOutMax=[]  DOutMin=[]  DOutMax=[]  NOutMin=[]  NOutMax=[]  SumOutMin=[]  SumOutMax=[]  SaturationOutMin=[]  SaturationOutMax=[]  PParamMin=[]  PParamMax=[]  IParamMin=[]  IParamMax=[]  DParamMin=[]  DParamMax=[]  NParamMin=[]  NParamMax=[]  KbParamMin=[]  KbParamMax=[]  KtParamMin=[]  KtParamMax=[]  KbOutMin=[]  KbOutMax=[]  KtOutMin=[]  KtOutMax=[]  IntegratorOutMin=[]  IntegratorOutMax=[]  FilterOutMin=[]  FilterOutMax=[]  SumI1OutMin=[]  SumI1OutMax=[]  SumI2OutMin=[]  SumI2OutMax=[]  SumI3OutMin=[]  SumI3OutMax=[]  SumI4OutMin=[]  SumI4OutMax=[]  SumDOutMin=[]  SumDOutMax=[]  DifferentiatorOutMin=[]  DifferentiatorOutMax=[]  FilterDiffOutCoefMin=[]  FilterDiffOutCoefMax=[]  ReciprocalOutMin=[]  ReciprocalOutMax=[]  SumDenOutMin=[]  SumDenOutMax=[]  SumNumOutMin=[]  SumNumOutMax=[]  DivideOutMin=[]  DivideOutMax=[]  UdiffTsProdOutMin=[]  UdiffTsProdOutMax=[]  NTsProdOutMin=[]  NTsProdOutMax=[]  UintegralTsProdOutMin=[]  UintegralTsProdOutMax=[]  UngainTsProdOutMin=[]  UngainTsProdOutMax=[]  ClampingZeroOutDataTypeStr=Inherit: Inherit via back propagation  ClampingZeroOutMin=[]  ClampingZeroOutMax=[]  FilterDenConstantOutDataTypeStr=Inherit: Inherit via back propagation  FilterDenConstantOutMin=[]  FilterDenConstantOutMax=[]  PCopyOutDataTypeStr=Inherit: Inherit via back propagation  PCopyOutMin=[]  PCopyOutMax=[]  NCopyOutDataTypeStr=Inherit: Inherit via back propagation  NCopyOutMin=[]  NCopyOutMax=[]  IntegratorContinuousStateAttributes=''  IntegratorStateMustResolveToSignalObject=off  IntegratorRTWStateStorageClass=Auto  FilterContinuousStateAttributes=''  FilterStateMustResolveToSignalObject=off  FilterRTWStateStorageClass=Auto  ParallelPVariant=InternalParameters  IdealPVariant=Disabled  IVariant=InternalParameters  DVariant=InternalParameters  IntegratorVariant=Discrete  SatVariant=Disabled  AWVariant=Passthrough  PCopyVariant=Disabled  TRVariant=Disabled  FdbkBlocksVariant=Forward  IdealPFdbkVariant=Disabled  SatFdbkVariant=Disabled  DerivativeFilterVariant=ForwardEulerFilter  NVariant=InternalParameters  NCopyVariant=Disabled  FilterICVariant=InternalICsFilter  IntegratorICVariant=InternalICs  ExternalResetVariant=Disabled  TRSumVariant=Passthrough  SumFdbkVariant=Disabled  SumVariant=Sum_PID  TsampFilterVariant=InternalTs  TsampNgainVariant=Passthrough  TsampIntegralVariant=Passthrough  ExternalSaturationOutDataTypeStr=Inherit: Same as second input
  Saturation3 : Saturate  UpperLimit=1800*80.4  LowerLimit=0
  Sum1 : Sum  Inputs=|+-
  Sum2 : Sum  Inputs=|++
  Torque3 : Scope  NumInputPorts=2
  kappa3 : Scope  NumInputPorts=2
  Out1 : Outport
  wires:
  Saturation3/1 -> Out1/1
  If Action Subsystem1/1(kappa_d) -> Merge/1
  If Action Subsystem2/1(kappa_d) -> Merge/3
  Gain/1 -> Sum2/2
  If/3 -> If Action Subsystem2/Action
  FxL2/1 -> If Action Subsystem/1(Fx), If Action Subsystem1/1(Fx), Gain/1, If Action Subsystem2/1(Fx)
  kappa_L2/1 -> kappa3/2, Sum1/2
  FzL2/1 -> If/1
  If Action Subsystem/1(kappa_d) -> Merge/2
  If/2 -> If Action Subsystem/Action
  If/1 -> If Action Subsystem1/Action
  Sum2/1 -> Torque3/2, Saturation3/1
  Sum1/1 -> PID Controller/1
  Merge/1 -> kappa3/1, Sum1/1
  PID Controller/1 -> Torque3/1, Sum2/1

== system launch_gate_exp/总驱动力矩制定/正常工况_高速衰减防抖/Subsystem1 ==
  v : Inport
  Add : Sum
  Constant : Constant  Value=200
  Constant1 : Constant  Value=50
  Constant2 : Constant  Value=5
  Divide : Product  Inputs=*/
  Gain : Gain  Gain=5000-200
  Sum : Sum  Inputs=|+-
  Out1 : Outport
  wires:
  Add/1 -> Out1/1
  Gain/1 -> Add/2
  Divide/1 -> Gain/1
  Constant2/1 -> Divide/2
  Sum/1 -> Divide/1
  v/1 -> Sum/2
  Constant1/1 -> Sum/1
  Constant/1 -> Add/1

== system launch_gate_exp/总驱动力矩制定/正常工况_高速衰减防抖/高速衰减冻结区 ==
  v : Inport
  Add : Sum
  Constant : Constant  Value=200
  Constant1 : Constant  Value=20
  Constant2 : Constant  Value=2
  Divide : Product  Inputs=*/
  Gain : Gain  Gain=1000-200
  Sum : Sum  Inputs=|+-
  Out1 : Outport
  wires:
  Constant/1 -> Add/1
  Constant1/1 -> Sum/1
  v/1 -> Sum/2
  Sum/1 -> Divide/1
  Constant2/1 -> Divide/2
  Divide/1 -> Gain/1
  Gain/1 -> Add/2
  Add/1 -> Out1/1

== system launch_gate_exp/质心侧偏角估计/Observer/Subsystem ==
  note: yhat[k|k-1]
  L[k] : Inport
  y[k] : Inport  Port=2
  C[k] : Inport  Port=3
  xhat[k|k-1] : Inport  Port=4
  D[k] : Inport  Port=5
  u[k] : Inport  Port=6
  Add : Sum  Inputs=+-
  Add1 : Sum
  C[k]*xhat[k|k-1] : Product  Multiplication=Matrix(*)
  D[k]*u[k] : Product  Multiplication=Matrix(*)
  Matrix Multiply : Product  Multiplication=Matrix(*)
  L*(y[k]-yhat[k|k-1]) : Outport
  wires:
  L[k]/1 -> Matrix Multiply/1
  y[k]/1 -> Add/1
  C[k]/1 -> C[k]*xhat[k|k-1]/1
  xhat[k|k-1]/1 -> C[k]*xhat[k|k-1]/2
  C[k]*xhat[k|k-1]/1 -> Add1/1
  D[k]/1 -> D[k]*u[k]/1
  u[k]/1 -> D[k]*u[k]/2
  D[k]*u[k]/1 -> Add1/2
  Add1/1 -> Add/2
  Add/1 -> Matrix Multiply/2
  Matrix Multiply/1 -> L*(y[k]-yhat[k|k-1])/1

== system launch_gate_exp/质心侧偏角滑模观测器估计/Subsystem/Subsystem ==
  error : Inport
  Abs : Abs  SaturateOnIntegerOverflow=off
  Discrete-Time Integrator : DiscreteIntegrator  SampleTime=-1  ICPrevOutput=DiscIntNeverNeededParam  ICPrevScaledInput=DiscIntNeverNeededParam
  Gain : Gain  Gain=K1
  Gain1 : Gain  Gain=K2
  Product : Product
  Sign : Signum
  Sqrt : Sqrt
  Sum : Sum  Inputs=|++
  v_STA : Outport
  wires:
  error/1 -> Abs/1, Sign/1
  Abs/1 -> Sqrt/1
  Sqrt/1 -> Product/1
  Sign/1 -> Gain1/1, Product/2
  Product/1 -> Gain/1
  Gain1/1 -> Discrete-Time Integrator/1
  Sum/1 -> v_STA/1
  Gain/1 -> Sum/1
  Discrete-Time Integrator/1 -> Sum/2

== system launch_gate_exp/驱动防滑模块/滑转率计算/Subsystem ==
  In1 : Inport
  In2 : Inport  Port=2
  In3 : Inport  Port=3
  Abs : Abs  SaturateOnIntegerOverflow=off
  Constant4 : Constant  Value=0.1
  Constant5 : Constant  Value=0.2
  Constant6 : Constant  Value=-1.2
  Constant7 : Constant  Value=1.2
  Logical Operator : Logic  Inputs=3  AllPortsSameDT=off  OutDataTypeStr=boolean
  Logical Operator1 : Logic  AllPortsSameDT=off  OutDataTypeStr=boolean
  Relational Operator : RelationalOperator  OutDataTypeStr=boolean  RndMeth=Simplest  InputSameDT=off
  Relational Operator1 : RelationalOperator  OutDataTypeStr=boolean  RndMeth=Simplest  InputSameDT=off
  Relational Operator2 : RelationalOperator  Operator=>  OutDataTypeStr=boolean  RndMeth=Simplest  InputSameDT=off
  Relational Operator3 : RelationalOperator  Operator=<  OutDataTypeStr=boolean  RndMeth=Simplest  InputSameDT=off
  slip_valid_fl : Outport
  wires:
  Logical Operator1/1 -> Logical Operator/3
  Constant4/1 -> Relational Operator/2
  Relational Operator/1 -> Logical Operator/1
  Constant7/1 -> Relational Operator3/2
  In3/1 -> Relational Operator3/1, Relational Operator2/1
  Abs/1 -> Relational Operator/1
  Constant5/1 -> Relational Operator1/2
  Relational Operator2/1 -> Logical Operator1/1
  Constant6/1 -> Relational Operator2/2
  In1/1 -> Abs/1
  Relational Operator3/1 -> Logical Operator1/2
  In2/1 -> Relational Operator1/1
  Relational Operator1/1 -> Logical Operator/2
  Logical Operator/1 -> slip_valid_fl/1

== system launch_gate_exp/驱动防滑模块/滑转率计算/Subsystem1 ==
  In1 : Inport
  In2 : Inport  Port=2
  In3 : Inport  Port=3
  Abs : Abs  SaturateOnIntegerOverflow=off
  Constant4 : Constant  Value=0.1
  Constant5 : Constant  Value=0.2
  Constant6 : Constant  Value=-1.2
  Constant7 : Constant  Value=1.2
  Logical Operator : Logic  Inputs=3  AllPortsSameDT=off  OutDataTypeStr=boolean
  Logical Operator1 : Logic  AllPortsSameDT=off  OutDataTypeStr=boolean
  Relational Operator : RelationalOperator  OutDataTypeStr=boolean  RndMeth=Simplest  InputSameDT=off
  Relational Operator1 : RelationalOperator  OutDataTypeStr=boolean  RndMeth=Simplest  InputSameDT=off
  Relational Operator2 : RelationalOperator  Operator=>  OutDataTypeStr=boolean  RndMeth=Simplest  InputSameDT=off
  Relational Operator3 : RelationalOperator  Operator=<  OutDataTypeStr=boolean  RndMeth=Simplest  InputSameDT=off
  slip_valid_fr : Outport
  wires:
  Logical Operator/1 -> slip_valid_fr/1
  Relational Operator1/1 -> Logical Operator/2
  In2/1 -> Relational Operator1/1
  Relational Operator3/1 -> Logical Operator1/2
  In1/1 -> Abs/1
  Constant6/1 -> Relational Operator2/2
  Relational Operator2/1 -> Logical Operator1/1
  Constant5/1 -> Relational Operator1/2
  Abs/1 -> Relational Operator/1
  In3/1 -> Relational Operator2/1, Relational Operator3/1
  Constant7/1 -> Relational Operator3/2
  Relational Operator/1 -> Logical Operator/1
  Constant4/1 -> Relational Operator/2
  Logical Operator1/1 -> Logical Operator/3

== system launch_gate_exp/驱动防滑模块/滑转率计算/Subsystem2 ==
  In1 : Inport
  In2 : Inport  Port=2
  In3 : Inport  Port=3
  Abs : Abs  SaturateOnIntegerOverflow=off
  Constant4 : Constant  Value=0.1
  Constant5 : Constant  Value=0.2
  Constant6 : Constant  Value=-1.2
  Constant7 : Constant  Value=1.2
  Logical Operator : Logic  Inputs=3  AllPortsSameDT=off  OutDataTypeStr=boolean
  Logical Operator1 : Logic  AllPortsSameDT=off  OutDataTypeStr=boolean
  Relational Operator : RelationalOperator  OutDataTypeStr=boolean  RndMeth=Simplest  InputSameDT=off
  Relational Operator1 : RelationalOperator  OutDataTypeStr=boolean  RndMeth=Simplest  InputSameDT=off
  Relational Operator2 : RelationalOperator  Operator=>  OutDataTypeStr=boolean  RndMeth=Simplest  InputSameDT=off
  Relational Operator3 : RelationalOperator  Operator=<  OutDataTypeStr=boolean  RndMeth=Simplest  InputSameDT=off
  slip_valid_rl : Outport
  wires:
  Logical Operator1/1 -> Logical Operator/3
  Constant4/1 -> Relational Operator/2
  Relational Operator/1 -> Logical Operator/1
  Constant7/1 -> Relational Operator3/2
  In3/1 -> Relational Operator3/1, Relational Operator2/1
  Abs/1 -> Relational Operator/1
  Constant5/1 -> Relational Operator1/2
  Relational Operator2/1 -> Logical Operator1/1
  Constant6/1 -> Relational Operator2/2
  In1/1 -> Abs/1
  Relational Operator3/1 -> Logical Operator1/2
  In2/1 -> Relational Operator1/1
  Relational Operator1/1 -> Logical Operator/2
  Logical Operator/1 -> slip_valid_rl/1

== system launch_gate_exp/驱动防滑模块/滑转率计算/Subsystem3 ==
  In1 : Inport
  In2 : Inport  Port=2
  In3 : Inport  Port=3
  Abs : Abs  SaturateOnIntegerOverflow=off
  Constant4 : Constant  Value=0.1
  Constant5 : Constant  Value=0.2
  Constant6 : Constant  Value=-1.2
  Constant7 : Constant  Value=1.2
  Logical Operator : Logic  Inputs=3  AllPortsSameDT=off  OutDataTypeStr=boolean
  Logical Operator1 : Logic  AllPortsSameDT=off  OutDataTypeStr=boolean
  Relational Operator : RelationalOperator  OutDataTypeStr=boolean  RndMeth=Simplest  InputSameDT=off
  Relational Operator1 : RelationalOperator  OutDataTypeStr=boolean  RndMeth=Simplest  InputSameDT=off
  Relational Operator2 : RelationalOperator  Operator=>  OutDataTypeStr=boolean  RndMeth=Simplest  InputSameDT=off
  Relational Operator3 : RelationalOperator  Operator=<  OutDataTypeStr=boolean  RndMeth=Simplest  InputSameDT=off
  slip_valid_rl : Outport
  wires:
  Logical Operator/1 -> slip_valid_rl/1
  Relational Operator1/1 -> Logical Operator/2
  In2/1 -> Relational Operator1/1
  Relational Operator3/1 -> Logical Operator1/2
  In1/1 -> Abs/1
  Constant6/1 -> Relational Operator2/2
  Relational Operator2/1 -> Logical Operator1/1
  Constant5/1 -> Relational Operator1/2
  Abs/1 -> Relational Operator/1
  In3/1 -> Relational Operator2/1, Relational Operator3/1
  Constant7/1 -> Relational Operator3/2
  Relational Operator/1 -> Logical Operator/1
  Constant4/1 -> Relational Operator/2
  Logical Operator1/1 -> Logical Operator/3

== system launch_gate_exp/Dugoff轮胎模型/alpha_lamda/alpha/fl ==
  vx : Inport
  vy : Inport  Port=2
  wz : Inport  Port=3
  delta_fl : Inport  Port=4
  Add2 : Sum
  Add3 : Sum  Inputs=+-
  Add4 : Sum  Inputs=-+
  Divide : Product  Inputs=/*
  Gain3 : Gain  Gain=2.043
  Gain4 : Gain  Gain=0.5*2.39
  Trigonometric Function : Trigonometry  Operator=atan
  alpha_fl : Outport
  wires:
  wz/1 -> Gain3/1, Gain4/1
  Add4/1 -> alpha_fl/1
  vy/1 -> Add2/1
  delta_fl/1 -> Add4/2
  vx/1 -> Add3/1
  Trigonometric Function/1 -> Add4/1
  Divide/1 -> Trigonometric Function/1
  Add3/1 -> Divide/1
  Add2/1 -> Divide/2
  Gain4/1 -> Add3/2
  Gain3/1 -> Add2/2

== system launch_gate_exp/Dugoff轮胎模型/alpha_lamda/alpha/fr ==
  vx : Inport
  vy : Inport  Port=2
  wz : Inport  Port=3
  delta_fr : Inport  Port=4
  Add2 : Sum
  Add3 : Sum
  Add4 : Sum  Inputs=-+
  Divide : Product  Inputs=/*
  Gain3 : Gain  Gain=2.043
  Gain4 : Gain  Gain=0.5*2.39
  Trigonometric Function : Trigonometry  Operator=atan
  alpha_fr : Outport
  wires:
  Gain3/1 -> Add2/2
  Add2/1 -> Divide/2
  Add3/1 -> Divide/1
  Divide/1 -> Trigonometric Function/1
  Trigonometric Function/1 -> Add4/1
  vx/1 -> Add3/1
  delta_fr/1 -> Add4/2
  vy/1 -> Add2/1
  Add4/1 -> alpha_fr/1
  wz/1 -> Gain4/1, Gain3/1
  Gain4/1 -> Add3/2

== system launch_gate_exp/Dugoff轮胎模型/alpha_lamda/alpha/rl ==
  vx : Inport
  vy : Inport  Port=2
  wz : Inport  Port=3
  Add2 : Sum  Inputs=+-
  Add3 : Sum  Inputs=+-
  Divide : Product  Inputs=/*
  Gain1 : Gain  Gain=-1
  Gain3 : Gain  Gain=1.362
  Gain4 : Gain  Gain=0.5*2.33
  Trigonometric Function : Trigonometry  Operator=atan
  alpha_rl : Outport
  wires:
  Gain3/1 -> Add2/2
  Add2/1 -> Divide/2
  Add3/1 -> Divide/1
  Divide/1 -> Trigonometric Function/1
  vx/1 -> Add3/1
  vy/1 -> Add2/1
  wz/1 -> Gain4/1, Gain3/1
  Trigonometric Function/1 -> Gain1/1
  Gain4/1 -> Add3/2
  Gain1/1 -> alpha_rl/1

== system launch_gate_exp/Dugoff轮胎模型/alpha_lamda/alpha/rr ==
  vx : Inport
  vy : Inport  Port=2
  wz : Inport  Port=3
  Add2 : Sum  Inputs=+-
  Add3 : Sum
  Divide : Product  Inputs=/*
  Gain2 : Gain  Gain=-1
  Gain3 : Gain  Gain=1.362
  Gain4 : Gain  Gain=0.5*2.33
  Trigonometric Function : Trigonometry  Operator=atan
  alpha_rr : Outport
  wires:
  Trigonometric Function/1 -> Gain2/1
  wz/1 -> Gain3/1, Gain4/1
  vy/1 -> Add2/1
  vx/1 -> Add3/1
  Divide/1 -> Trigonometric Function/1
  Add3/1 -> Divide/1
  Add2/1 -> Divide/2
  Gain3/1 -> Add2/2
  Gain4/1 -> Add3/2
  Gain2/1 -> alpha_rr/1

== system launch_gate_exp/Dugoff轮胎模型/alpha_lamda/lamda/fl ==
  w_fl : Inport
  wz : Inport  Port=2
  vx : Inport  Port=3
  vy : Inport  Port=4
  delta_fl : Inport  Port=5
  Add1 : Sum  Inputs=-+
  Add2 : Sum
  Add3 : Sum
  Add4 : Sum  Inputs=+-
  Constant1 : Constant  Value=0.834
  Divide1 : Product  Inputs=**
  Divide2 : Product  Inputs=**
  Divide3 : Product  Inputs=**
  Divide4 : Product  Inputs=/*
  Divide5 : Product  Inputs=*/
  Fcn1 : Fcn  Expr=u+(u==0)*eps
  Gain2 : Gain  Gain=0.5*2.39
  Gain3 : Gain  Gain=2.043
  Saturation : Saturate  UpperLimit=1  LowerLimit=-1
  Switch : Switch  Criteria=u2 > Threshold  SaturateOnIntegerOverflow=off  InputSameDT=off
  Trigonometric Function1 : Trigonometry
  Trigonometric Function2 : Trigonometry  Operator=cos
  lamda_fl : Outport
  wires:
  Switch/1 -> Saturation/1
  Add3/1 -> Add4/2, Divide5/2  "Vwx_fl"
  Add4/1 -> Switch/2, Divide4/2, Divide5/1
  Divide4/1 -> Switch/1
  Divide5/1 -> Switch/3
  Fcn1/1 -> Divide4/1
  vx/1 -> Add1/2
  Gain2/1 -> Add1/1
  wz/1 -> Gain3/1, Gain2/1
  Add1/1 -> Divide1/1
  delta_fl/1 -> Trigonometric Function2/1, Trigonometric Function1/1
  Trigonometric Function2/1 -> Divide1/2
  vy/1 -> Add2/2
  Gain3/1 -> Add2/1
  Add2/1 -> Divide2/1
  Trigonometric Function1/1 -> Divide2/2
  Divide1/1 -> Add3/1
  Divide2/1 -> Add3/2
  w_fl/1 -> Divide3/1
  Constant1/1 -> Divide3/2
  Divide3/1 -> Add4/1, Fcn1/1  "w*I_tire"
  Saturation/1 -> lamda_fl/1

== system launch_gate_exp/Dugoff轮胎模型/alpha_lamda/lamda/fr ==
  w_fr : Inport
  wz : Inport  Port=2
  vx : Inport  Port=3
  vy : Inport  Port=4
  delta_fr : Inport  Port=5
  Add1 : Sum
  Add2 : Sum
  Add3 : Sum
  Add4 : Sum  Inputs=+-
  Constant1 : Constant  Value=0.834
  Divide1 : Product  Inputs=**
  Divide2 : Product  Inputs=**
  Divide3 : Product  Inputs=**
  Divide4 : Product  Inputs=/*
  Divide5 : Product  Inputs=*/
  Fcn1 : Fcn  Expr=u+(u==0)*eps
  Gain2 : Gain  Gain=0.5*2.39
  Gain3 : Gain  Gain=2.043
  Saturation : Saturate  UpperLimit=1  LowerLimit=-1
  Switch : Switch  Criteria=u2 > Threshold  SaturateOnIntegerOverflow=off  InputSameDT=off
  Trigonometric Function1 : Trigonometry
  Trigonometric Function2 : Trigonometry  Operator=cos
  lamda_fr : Outport
  wires:
  Saturation/1 -> lamda_fr/1
  vx/1 -> Add1/2
  Gain2/1 -> Add1/1
  wz/1 -> Gain3/1, Gain2/1
  Add1/1 -> Divide1/1
  delta_fr/1 -> Trigonometric Function2/1, Trigonometric Function1/1
  Trigonometric Function2/1 -> Divide1/2
  vy/1 -> Add2/2
  Gain3/1 -> Add2/1
  Add2/1 -> Divide2/1
  Trigonometric Function1/1 -> Divide2/2
  Divide1/1 -> Add3/1
  Divide2/1 -> Add3/2
  w_fr/1 -> Divide3/1
  Constant1/1 -> Divide3/2
  Divide3/1 -> Fcn1/1, Add4/1  "w*I_tire"
  Fcn1/1 -> Divide4/1
  Divide5/1 -> Switch/3
  Divide4/1 -> Switch/1
  Add4/1 -> Divide5/1, Divide4/2, Switch/2
  Add3/1 -> Divide5/2, Add4/2  "Vwx_fr"
  Switch/1 -> Saturation/1

== system launch_gate_exp/Dugoff轮胎模型/alpha_lamda/lamda/rl ==
  w_rl : Inport
  wz : Inport  Port=2
  vx : Inport  Port=3
  Add1 : Sum  Inputs=-+
  Add4 : Sum  Inputs=+-
  Constant1 : Constant  Value=0.94
  Divide3 : Product  Inputs=**
  Divide4 : Product  Inputs=/*
  Divide5 : Product  Inputs=*/
  Fcn1 : Fcn  Expr=u+(u==0)*eps
  Gain2 : Gain  Gain=0.5*2.33
  Saturation : Saturate  UpperLimit=1  LowerLimit=-1
  Switch : Switch  Criteria=u2 > Threshold  SaturateOnIntegerOverflow=off  InputSameDT=off
  lamda_rl : Outport
  wires:
  Saturation/1 -> lamda_rl/1
  vx/1 -> Add1/2
  Gain2/1 -> Add1/1
  wz/1 -> Gain2/1
  w_rl/1 -> Divide3/1
  Constant1/1 -> Divide3/2
  Divide3/1 -> Fcn1/1, Add4/1  "w*I_tire"
  Fcn1/1 -> Divide4/1
  Divide5/1 -> Switch/3
  Divide4/1 -> Switch/1
  Add4/1 -> Divide5/1, Divide4/2, Switch/2
  Add1/1 -> Divide5/2, Add4/2
  Switch/1 -> Saturation/1

== system launch_gate_exp/Dugoff轮胎模型/alpha_lamda/lamda/rr ==
  w_rr : Inport
  wz : Inport  Port=2
  vx : Inport  Port=3
  Add1 : Sum
  Add4 : Sum  Inputs=+-
  Constant1 : Constant  Value=0.94
  Divide3 : Product  Inputs=**
  Divide4 : Product  Inputs=/*
  Divide5 : Product  Inputs=*/
  Fcn1 : Fcn  Expr=u+(u==0)*eps
  Gain2 : Gain  Gain=0.5*2.33
  Saturation : Saturate  UpperLimit=1  LowerLimit=-1
  Switch : Switch  Criteria=u2 > Threshold  SaturateOnIntegerOverflow=off  InputSameDT=off
  lamda_rr : Outport
  wires:
  Saturation/1 -> lamda_rr/1
  Switch/1 -> Saturation/1
  Constant1/1 -> Divide3/2
  w_rr/1 -> Divide3/1
  wz/1 -> Gain2/1
  Gain2/1 -> Add1/1
  vx/1 -> Add1/2
  Divide3/1 -> Fcn1/1, Add4/1  "w*I_tire"
  Fcn1/1 -> Divide4/1
  Divide5/1 -> Switch/3
  Divide4/1 -> Switch/1
  Add4/1 -> Divide5/1, Divide4/2, Switch/2
  Add1/1 -> Divide5/2, Add4/2  "Vwx_rr"
